simulink model "LunarMicrogridA"  (R2026b)
settings: Solver=ode23t  StopTime=simulation.timeSim  MaxStep=1/(5*solarPlant.converterSwitchingFrequency)  AbsTol=1e-3
PreLoadFcn:
  | run('LunarMicrogridA_Data');
undefined symbols (not defined in the file or in its folder): battery, bms, bmsController, boostController, connectedLoad, dcVoltage, lunarCase, maxSoC, maxVdc, minIrrad, minSoC, minVdc, olTime, sensor, solarPanel, solarPlant
libraries: fl_lib x17, nesl_utility x15, simulink x13, ee_lib x6, eePwmGenerator x3, simulink_extras x2, batteryecm_lib x1
(part 2 of 2)

== system LunarMicrogridA/PV Control/Maximum Power Point ==
  "IL " : Inport
  "Vo " : Inport  Port=2
  Vpv : Inport  Port=3
  Ipv : Inport  Port=4
  Enable : EnablePort  StatesWhenEnabling=reset
  MPPT : Subsystem
  MPPT Subsystem : Subsystem  TreatAsAtomicUnit=on
  Rate Transition : RateTransition  OutPortSampleTime=0.02
  ZOH/4 : ZeroOrderHold  SampleTime=solarPlant.timeMPPT
  Gmpp : Outport
  Vmpp : Outport  Port=2
  wires:
  ZOH/4/1 -> MPPT/2(Vpv)
  Rate Transition/1 -> MPPT/1(Ipv)
  MPPT/1(Vmpp) -> Vmpp/1, MPPT Subsystem/1(VpvRef)
  "Vo "/1 -> MPPT Subsystem/4("Vo ")
  Ipv/1 -> Rate Transition/1
  Vpv/1 -> MPPT Subsystem/2(Vpv), ZOH/4/1
  MPPT Subsystem/1(G) -> Gmpp/1
  "IL "/1 -> MPPT Subsystem/3(IL)

== system LunarMicrogridA/PV Control/PV Isolate ==
  Enable : EnablePort  StatesWhenEnabling=reset
  Constant : Constant  Value=0
  Gain : Gain
  Rate Transition : RateTransition
  Gmpp : Outport
  wires:
  Constant/1 -> Gain/1
  Gain/1 -> Rate Transition/1
  Rate Transition/1 -> Gmpp/1

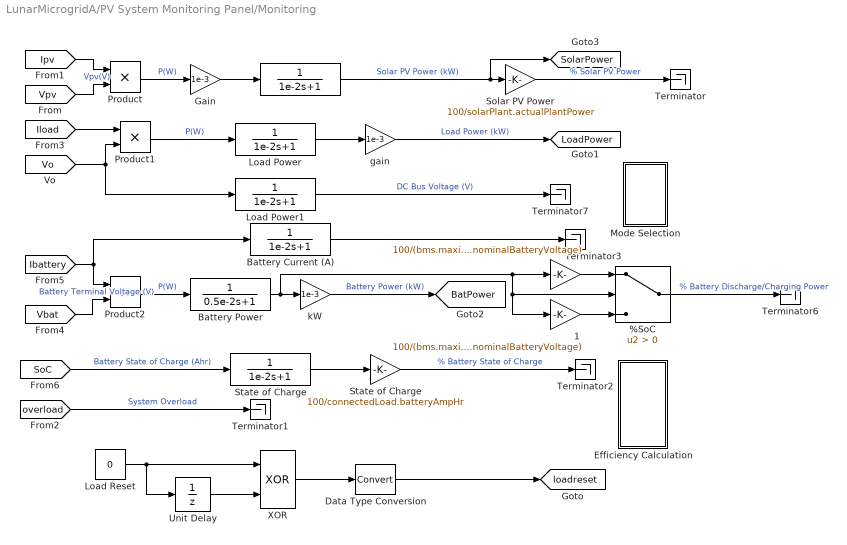
== system LunarMicrogridA/PV System Monitoring Panel/Monitoring ==
  " " : Gain  Gain=100/(bms.maximumChargingCurrentLimit*battery.nominalBatteryVoltage)
  "  " : TransferFcn  Denominator=[1e-2 1]
  " 1" : Gain  Gain=100/(bms.maximumDisChargingCurrent*battery.nominalBatteryVoltage)
  " State of Charge" : Gain  Gain=100/connectedLoad.batteryAmpHr
  %SoC : Switch  Criteria=u2 > Threshold  SaturateOnIntegerOverflow=off  InputSameDT=off
  Battery Current (A) : TransferFcn  Denominator=[1e-2 1]
  Battery Power : TransferFcn  Denominator=[0.5e-2 1]
  Data Type Conversion : DataTypeConversion  SaturateOnIntegerOverflow=off  RndMeth=Floor
  Efficiency Calculation : Subsystem
  Gain : Gain  Gain=1e-3
  Load Power : TransferFcn  Denominator=[1e-2 1]
  Load Power1 : TransferFcn  Denominator=[1e-2 1]
  Load Reset : Constant  Value=0
  Mode Selection : Subsystem
  Product : Product
  Product1 : Product
  Product2 : Product
  Solar PV Power : Gain  Gain=100/solarPlant.actualPlantPower
  State of Charge : TransferFcn  Denominator=[1e-2 1]
  Terminator{,1..3,6..7} (6 alike) : Terminator
  Unit Delay : UnitDelay  SampleTime=1e-3
  XOR : Logic  Operator=XOR  IconShape=distinctive  AllPortsSameDT=off  OutDataTypeStr=boolean
  gain : Gain  Gain=1e-3
  kW : Gain  Gain=1e-3
  tag scope: BatPower=global, LoadPower=global, SolarPower=global, loadreset=global
  wires:
  [Vpv] -> Product/2  "Vpv(V)"
  Load Power/1 -> gain/1
  Product1/1 -> Load Power/1  "P(W)"
  [Vbat] -> Product2/2  "Battery Terminal Voltage (V)"
  [Iload] -> Product1/1
  Battery Power/1 -> kW/1, " 1"/1, %SoC/2, " "/1
  "  "/1 -> [SolarPower], Solar PV Power/1  "Solar PV Power (kW)"
  [Ibattery] -> Product2/1, Battery Current (A)/1
  Product2/1 -> Battery Power/1  "P(W)"
  [Ipv] -> Product/1
  [Vo] -> Product1/2, Load Power1/1
  Product/1 -> Gain/1  "P(W)"
  [SoC] -> State of Charge/1  "Battery State of Charge (Ahr)"
  Solar PV Power/1 -> Terminator/1  "% Solar PV Power"
  gain/1 -> [LoadPower]  "Load Power (kW)"
  kW/1 -> [BatPower]  "Battery Power (kW)"
  State of Charge/1 -> " State of Charge"/1
  " State of Charge"/1 -> Terminator2/1  "% Battery State of Charge"
  " "/1 -> %SoC/1
  " 1"/1 -> %SoC/3
  %SoC/1 -> Terminator6/1  "% Battery Discharge/Charging Power"
  Battery Current (A)/1 -> Terminator3/1
  Gain/1 -> "  "/1
  Load Power1/1 -> Terminator7/1  "DC Bus Voltage (V)"
  [overload] -> Terminator1/1  "System Overload"
  XOR/1 -> Data Type Conversion/1
  Load Reset/1 -> XOR/1, Unit Delay/1
  Unit Delay/1 -> XOR/2
  Data Type Conversion/1 -> [loadreset]

== system LunarMicrogridA/Solar Plant/Solar Panel ==
  Current-Controlled Current Source : fl_lib/Electrical/Electrical Sources/Current-Controlled Current Source  K=-1*(solarPanel.numParallelCell-1)  i1_specify=off  i1_priority=None  i1=0 A  i1_nominal_specify=off  i1_nominal_value=1  i1_nominal_unit=A  i2_specify=off  i2_priority=None  i2=0 A  i2_nominal_specify=off  i2_nominal_value=1  i2_nominal_unit=A
  Solar Cell : ee_lib/Sources/Solar Cell  prm=1  Isc=solarPanel.shortCircuitCurrentPV/solarPanel.numParallelCell A  Voc=solarPanel.openCircuitVoltagePV/solarPanel.numSeriesCell V  Is=1e-6 A  Is2=0 A  Iph=7.34 A  Ir0=solarPanel.irradianceMeasurement W/m^2  ec=solarPanel.qualityFactor  N2=2  Rs=solarPanel.seriesResistance Ohm  Rp=inf Ohm  N_series=solarPanel.numSeriesCell-1  N_parallel=1  TIPH1=solarPanel.currentTemperatureCoeff 1/K  EG=1.11 eV  TXIS1=solarPanel.temperatureExponent  TXIS2=3  TRS1=0  TRP1=0  Tmeas=solarPanel.temperatureMeasurement degC  TFIXED=environment.temperature degC  thermal_mass=100 J/K  initial_temperature=25 degC
  Ir : PMIOPort  Side=Left
  + : PMIOPort  Port=2  Side=Right
  - : PMIOPort  Port=3  Side=Right
  connections:
  Current-Controlled Current Source/LConn2 -- -/RConn1 -- Solar Cell/RConn1
  Ir/RConn1 -- Solar Cell/LConn1
  Current-Controlled Current Source/LConn1 -- Solar Cell/LConn2
  Current-Controlled Current Source/RConn1 -- Current-Controlled Current Source/RConn2 -- +/RConn1

== system LunarMicrogridA/Battery Management Control/Battery Charging/Current control ==
  e : Inport
  1/T : Gain  Gain=1/bms.chargeCurrentZeroTimeConst
  Integrator : Integrator  LimitOutput=on  UpperSaturationLimit=1.3  LowerSaturationLimit=-1.3
  Kp : Gain  Gain=bms.chargeCurrentGain
  Saturation : Saturate  UpperLimit=1.5  LowerLimit=-1.5
  Sum7 : Sum  Inputs=|++
  u : Outport  VectorParamsAs1DForOutWhenUnconnected=off
  wires:
  Integrator/1 -> Sum7/2
  Saturation/1 -> u/1
  Sum7/1 -> Saturation/1
  e/1 -> Kp/1
  Kp/1 -> 1/T/1, Sum7/1
  1/T/1 -> Integrator/1

== system LunarMicrogridA/Battery Management Control/Battery Charging/Voltage control ==
  e : Inport
  1/T : Gain  Gain=1/bmsController.chosenChargeVoltageZeroTimeConst
  Integrator : Integrator  LimitOutput=on  UpperSaturationLimit=bms.maximumChargingCurrentLimit  LowerSaturationLimit=-1*bms.maximumChargingCurrentLimit
  Kp : Gain  Gain=bmsController.chosenChargeVoltageGain
  Saturation : Saturate  UpperLimit=bms.maximumChargingCurrentLimit  LowerLimit=-1*bms.maximumChargingCurrentLimit
  Sum7 : Sum  Inputs=|++
  u : Outport  VectorParamsAs1DForOutWhenUnconnected=off
  wires:
  Integrator/1 -> Sum7/2
  Saturation/1 -> u/1
  e/1 -> Kp/1
  Kp/1 -> 1/T/1, Sum7/1
  1/T/1 -> Integrator/1
  Sum7/1 -> Saturation/1

== system LunarMicrogridA/Battery Management Control/Battery Discharging/Current control ==
  e : Inport
  1/T : Gain  Gain=1/bms.dischargeCurrentZeroTimeConst
  Integrator : Integrator  InitialCondition=1  LimitOutput=on  UpperSaturationLimit=1  LowerSaturationLimit=-0.5
  Kp : Gain  Gain=bms.dischargeCurrentGain
  Saturation : Saturate  UpperLimit=1  LowerLimit=-1
  Sum7 : Sum  Inputs=|++
  u : Outport  VectorParamsAs1DForOutWhenUnconnected=off
  wires:
  Integrator/1 -> Sum7/2
  Saturation/1 -> u/1
  Sum7/1 -> Saturation/1
  e/1 -> Kp/1
  Kp/1 -> 1/T/1, Sum7/1
  1/T/1 -> Integrator/1

== system LunarMicrogridA/Battery Management Control/Battery Discharging/Voltage control ==
  e : Inport
  1/T : Gain  Gain=1/bmsController.chosenDischargeVoltageZeroTimeConst
  Integrator : Integrator  LimitOutput=on  UpperSaturationLimit=bms.maximumDisChargingCurrent  LowerSaturationLimit=-1*bms.maximumDisChargingCurrent
  Kp : Gain  Gain=bmsController.chosenDischargeVoltageGain
  Saturation : Saturate  UpperLimit=bms.maximumDisChargingCurrent  LowerLimit=-1*bms.maximumDisChargingCurrent
  Sum7 : Sum  Inputs=|++
  u : Outport  VectorParamsAs1DForOutWhenUnconnected=off
  wires:
  Integrator/1 -> Sum7/2
  Saturation/1 -> u/1
  e/1 -> Kp/1
  Kp/1 -> 1/T/1, Sum7/1
  1/T/1 -> Integrator/1
  Sum7/1 -> Saturation/1

== system LunarMicrogridA/PV Control/Constant Voltage/Current control ==
  e : Inport
  Integrator : Integrator  LimitOutput=on  UpperSaturationLimit=1.5  LowerSaturationLimit=-1.5
  Ki : Gain  Gain=1/boostController.mppCurrentZeroTimeConst
  Kp : Gain  Gain=boostController.mppCurrentGain
  Saturation : Saturate  UpperLimit=1.5  LowerLimit=-1.5
  Sum7 : Sum  Inputs=|++
  u : Outport  VectorParamsAs1DForOutWhenUnconnected=off
  wires:
  Integrator/1 -> Sum7/2
  Saturation/1 -> u/1
  Sum7/1 -> Saturation/1
  e/1 -> Kp/1
  Kp/1 -> Ki/1, Sum7/1
  Ki/1 -> Integrator/1

== system LunarMicrogridA/PV Control/Constant Voltage/Voltage control ==
  e : Inport
  1/T : Gain  Gain=1/boostController.mppVoltageZeroTimeConst
  Integrator : Integrator  LimitOutput=on  UpperSaturationLimit=boostController.mppVoltageLoopMax  LowerSaturationLimit=boostController.mppVoltageLoopMin
  Kp : Gain  Gain=boostController.mppVoltageGain
  Saturation : Saturate  UpperLimit=boostController.mppVoltageLoopMax  LowerLimit=boostController.mppVoltageLoopMin
  Sum7 : Sum  Inputs=|++
  u : Outport  VectorParamsAs1DForOutWhenUnconnected=off
  wires:
  Integrator/1 -> Sum7/2
  Saturation/1 -> u/1
  Sum7/1 -> Saturation/1
  e/1 -> Kp/1
  Kp/1 -> 1/T/1, Sum7/1
  1/T/1 -> Integrator/1

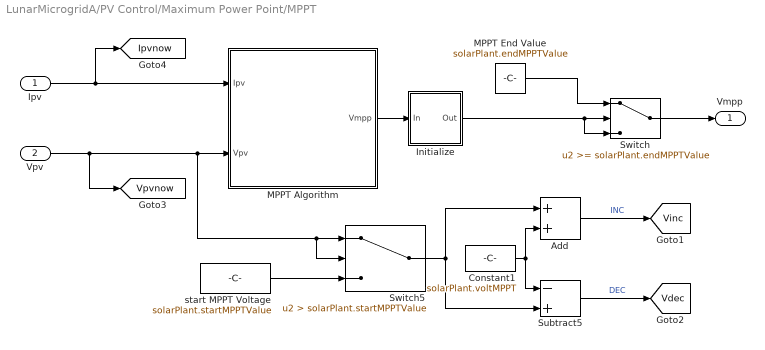
== system LunarMicrogridA/PV Control/Maximum Power Point/MPPT ==
  Ipv : Inport
  Vpv : Inport  Port=2
  Add : Sum
  Constant1 : Constant  Value=solarPlant.voltMPPT
  Initialize : Subsystem
  MPPT Algorithm : Subsystem  Variant=on
  MPPT End Value : Constant  Value=solarPlant.endMPPTValue
  Subtract5 : Sum  Inputs=-+
  Switch : Switch  Threshold=solarPlant.endMPPTValue  SaturateOnIntegerOverflow=off  InputSameDT=off
  Switch5 : Switch  Criteria=u2 > Threshold  Threshold=solarPlant.startMPPTValue  SaturateOnIntegerOverflow=off  InputSameDT=off
  start MPPT Voltage : Constant  Value=solarPlant.startMPPTValue
  Vmpp : Outport  VectorParamsAs1DForOutWhenUnconnected=off
  tag scope: Ipvnow=global, Vdec=global, Vinc=global, Vpvnow=global
  wires:
  Switch5/1 -> Add/1, Subtract5/2
  Add/1 -> [Vinc]  "INC"
  start MPPT Voltage/1 -> Switch5/3
  Vpv/1 -> [Vpvnow], Switch5/2, Switch5/1, MPPT Algorithm/2(Vpv)
  Constant1/1 -> Add/2, Subtract5/1
  Subtract5/1 -> [Vdec]  "DEC"
  Ipv/1 -> [Ipvnow], MPPT Algorithm/1(Ipv)
  MPPT Algorithm/1(Vmpp) -> Initialize/1(In)
  Initialize/1(Out) -> Switch/3, Switch/2
  Switch/1 -> Vmpp/1
  MPPT End Value/1 -> Switch/1

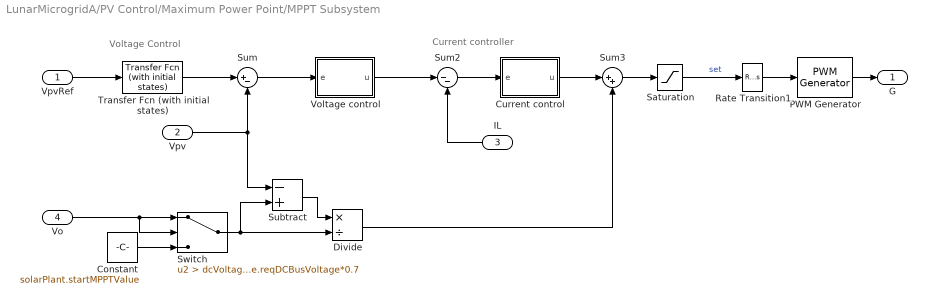
== system LunarMicrogridA/PV Control/Maximum Power Point/MPPT Subsystem ==
  note: Current controller
  note: Voltage Control
  VpvRef : Inport
  Vpv : Inport  Port=2
  IL : Inport  Port=3
  "Vo " : Inport  Port=4
  Constant : Constant  Value=solarPlant.startMPPTValue
  Current control : Subsystem
  Divide : Product  Inputs=*/
  PWM Generator : eePwmGenerator/PWM Generator  CarrCount=Up  Tper=1/solarPlant.converterSwitchingFrequency  Tdelay=0  Ts=1/(10*solarPlant.converterSwitchingFrequency)
  Rate Transition1 : RateTransition  OutPortSampleTime=1/(10*solarPlant.converterSwitchingFrequency)
  Saturation : Saturate  UpperLimit=1  LowerLimit=0
  Subtract : Sum  Inputs=-+
  Sum : Sum  Inputs=|+-
  Sum2 : Sum  Inputs=|--
  Sum3 : Sum  Inputs=|++
  Switch : Switch  Criteria=u2 > Threshold  Threshold=dcVoltage.reqDCBusVoltage*0.7  SaturateOnIntegerOverflow=off  InputSameDT=off
  Transfer Fcn (with initial states) : simulink_extras/Additional Linear/Transfer Fcn (with initial states)  N=[1]  D=[0.00001 1]  X0=solarPlant.startMPPTValue
  Voltage control : Subsystem
  G : Outport
  wires:
  Subtract/1 -> Divide/1
  Voltage control/1(u) -> Sum2/1
  Current control/1(u) -> Sum3/1
  Sum2/1 -> Current control/1(e)
  "Vo "/1 -> Switch/2, Switch/1
  VpvRef/1 -> Transfer Fcn (with initial states)/1
  Constant/1 -> Switch/3
  Switch/1 -> Divide/2, Subtract/2
  Vpv/1 -> Subtract/1, Sum/2
  Saturation/1 -> Rate Transition1/1  "set"
  Rate Transition1/1 -> PWM Generator/1
  PWM Generator/1 -> G/1
  Divide/1 -> Sum3/2
  Sum/1 -> Voltage control/1(e)
  IL/1 -> Sum2/2
  Transfer Fcn (with initial states)/1 -> Sum/1
  Sum3/1 -> Saturation/1

== system LunarMicrogridA/PV System Monitoring Panel/Monitoring/Efficiency Calculation ==
  Abs : Abs  SaturateOnIntegerOverflow=off
  Add : Sum
  Add1 : Sum
  Constant : Constant  Value=100e3
  Constant1 : Constant  Value=100e3
  Divide : Product  Inputs=/*
  Divide1 : Product  Inputs=/*
  Gain : Gain  Gain=100
  Switch : Switch  Criteria=u2 > Threshold  SaturateOnIntegerOverflow=off  InputSameDT=off
  Switch1 : Switch  Criteria=u2 > Threshold  SaturateOnIntegerOverflow=off  InputSameDT=off
  Switch2 : Switch  Criteria=u2 > Threshold  SaturateOnIntegerOverflow=off  InputSameDT=off
  Terminator : Terminator
  wires:
  [BatPower] -> Abs/1, Add/2, Switch/2
  [LoadPower] -> Add/1
  [SolarPower] -> Switch1/1, Switch1/2, Add1/2
  Constant/1 -> Switch1/3
  Switch1/1 -> Divide/1
  Add/1 -> Divide/2
  Abs/1 -> Add1/1
  [LoadPower] -> Divide1/2
  Add1/1 -> Switch2/2, Switch2/1
  Constant1/1 -> Switch2/3
  Switch2/1 -> Divide1/1
  Divide/1 -> Switch/1
  Divide1/1 -> Switch/3
  Switch/1 -> Gain/1
  Gain/1 -> Terminator/1  "% Efficiency"

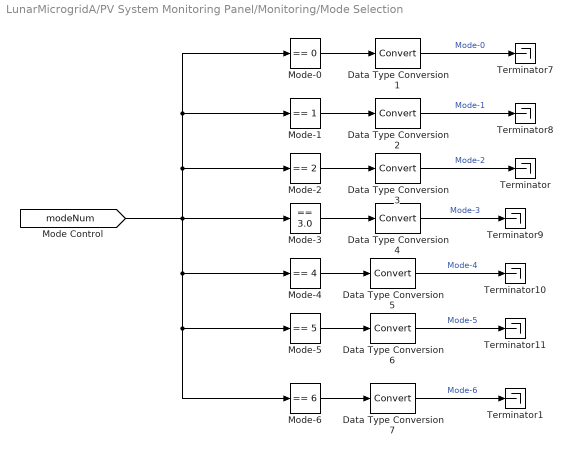
== system LunarMicrogridA/PV System Monitoring Panel/Monitoring/Mode Selection ==
  Data Type Conversion{1..7} (7 alike) : DataTypeConversion  SaturateOnIntegerOverflow=off  RndMeth=Floor
  Mode-0 : simulink/Logic and Bit Operations/Compare To Constant  relop===  const=0  OutDataTypeStr=boolean
  Mode-1 : simulink/Logic and Bit Operations/Compare To Constant  relop===  const=1  OutDataTypeStr=boolean
  Mode-2 : simulink/Logic and Bit Operations/Compare To Constant  relop===  const=2  OutDataTypeStr=boolean
  Mode-3 : simulink/Logic and Bit Operations/Compare To Constant  relop===  const=3.0  OutDataTypeStr=boolean
  Mode-4 : simulink/Logic and Bit Operations/Compare To Constant  relop===  const=4  OutDataTypeStr=boolean
  Mode-5 : simulink/Logic and Bit Operations/Compare To Constant  relop===  const=5  OutDataTypeStr=boolean
  Mode-6 : simulink/Logic and Bit Operations/Compare To Constant  relop===  const=6  OutDataTypeStr=boolean
  Terminator{,1,7..11} (7 alike) : Terminator
  wires:
  Mode-0/1 -> Data Type Conversion1/1
  Mode-3/1 -> Data Type Conversion4/1
  [modeNum] -> Mode-3/1, Mode-4/1, Mode-5/1, Mode-6/1, Mode-2/1, Mode-1/1, Mode-0/1
  Mode-4/1 -> Data Type Conversion5/1
  Mode-1/1 -> Data Type Conversion2/1
  Mode-2/1 -> Data Type Conversion3/1
  Mode-5/1 -> Data Type Conversion6/1
  Mode-6/1 -> Data Type Conversion7/1
  Data Type Conversion1/1 -> Terminator7/1  "Mode-0"
  Data Type Conversion2/1 -> Terminator8/1  "Mode-1"
  Data Type Conversion3/1 -> Terminator/1  "Mode-2"
  Data Type Conversion4/1 -> Terminator9/1  "Mode-3"
  Data Type Conversion5/1 -> Terminator10/1  "Mode-4"
  Data Type Conversion6/1 -> Terminator11/1  "Mode-5"
  Data Type Conversion7/1 -> Terminator1/1  "Mode-6"

== system LunarMicrogridA/PV Control/Maximum Power Point/MPPT/Initialize ==
  In : Inport
  Constant : Constant  Value=solarPlant.startMPPTValue
  Constant2 : Constant
  Integrator : Integrator
  Switch1 : Switch  Criteria=u2 > Threshold  Threshold=solarPlant.startMPPTValue  SaturateOnIntegerOverflow=off  InputSameDT=off
  Switch2 : Switch  Criteria=u2 > Threshold  Threshold=solarPlant.timeMPPT  SaturateOnIntegerOverflow=off  InputSameDT=off
  Out : Outport
  wires:
  Constant/1 -> Switch1/3
  Switch1/1 -> Switch2/1
  In/1 -> Switch1/2, Switch1/1
  Switch2/1 -> Out/1
  Constant2/1 -> Integrator/1
  [Vpvnow] -> Switch2/3
  Integrator/1 -> Switch2/2

== system LunarMicrogridA/PV Control/Maximum Power Point/MPPT/MPPT Algorithm ==
  Ipv : Inport
  Vpv : Inport  Port=2
  IncrementalConductance : Subsystem  VariantControl=incrementalConductance
  PerturbationAndObsrvation : Subsystem  VariantControl=perturbationAndObservation
  Vmpp : Outport  VectorParamsAs1DForOutWhenUnconnected=off

== system LunarMicrogridA/PV Control/Maximum Power Point/MPPT Subsystem/Current control ==
  e : Inport
  Integrator : Integrator  InitialCondition=1  LimitOutput=on  UpperSaturationLimit=1  LowerSaturationLimit=-0.5
  Ki : Gain  Gain=1/boostController.mppCurrentZeroTimeConst
  Kp : Gain  Gain=boostController.mppCurrentGain
  Saturation : Saturate  UpperLimit=1  LowerLimit=-0.3
  Sum7 : Sum  Inputs=|++
  u : Outport  VectorParamsAs1DForOutWhenUnconnected=off
  wires:
  Integrator/1 -> Sum7/2
  Saturation/1 -> u/1
  Sum7/1 -> Saturation/1
  e/1 -> Kp/1
  Kp/1 -> Ki/1, Sum7/1
  Ki/1 -> Integrator/1

== system LunarMicrogridA/PV Control/Maximum Power Point/MPPT Subsystem/Voltage control ==
  e : Inport
  1/T : Gain  Gain=1/boostController.mppVoltageZeroTimeConst
  Integrator : Integrator  LimitOutput=on  UpperSaturationLimit=boostController.mppVoltageLoopMax  LowerSaturationLimit=boostController.mppVoltageLoopMin
  Kp : Gain  Gain=boostController.mppVoltageGain
  Saturation : Saturate  UpperLimit=boostController.mppVoltageLoopMax  LowerLimit=boostController.mppVoltageLoopMin
  Sum7 : Sum  Inputs=|++
  u : Outport  VectorParamsAs1DForOutWhenUnconnected=off
  wires:
  Integrator/1 -> Sum7/2
  Saturation/1 -> u/1
  Sum7/1 -> Saturation/1
  e/1 -> Kp/1
  Kp/1 -> 1/T/1, Sum7/1
  1/T/1 -> Integrator/1

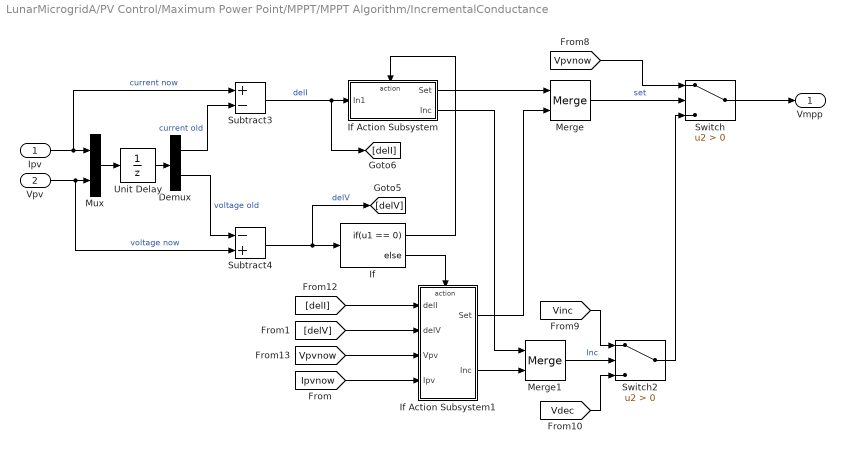
== system LunarMicrogridA/PV Control/Maximum Power Point/MPPT/MPPT Algorithm/IncrementalConductance ==
  Ipv : Inport
  Vpv : Inport  Port=2
  Demux : Demux  Outputs=2
  If : If  IfExpression=u1 == 0
  If Action Subsystem : Subsystem  TreatAsAtomicUnit=on
  If Action Subsystem1 : Subsystem  TreatAsAtomicUnit=on
  Merge : Merge
  Merge1 : Merge
  Mux : Mux  Inputs=2
  Subtract3 : Sum  Inputs=+-
  Subtract4 : Sum  Inputs=-+
  Switch : Switch  Criteria=u2 > Threshold  SaturateOnIntegerOverflow=off  InputSameDT=off
  Switch2 : Switch  Criteria=u2 > Threshold  SaturateOnIntegerOverflow=off  InputSameDT=off
  Unit Delay : UnitDelay  InitialCondition=solarPlant.startMPPTValue  SampleTime=solarPlant.timeMPPT
  Vmpp : Outport  VectorParamsAs1DForOutWhenUnconnected=off
  wires:
  Merge1/1 -> Switch2/2  "Inc"
  [Vpvnow] -> Switch/1
  If Action Subsystem1/2(Inc) -> Merge1/2
  If Action Subsystem/2(Inc) -> Merge1/1
  If/2 -> If Action Subsystem1/Action
  If Action Subsystem/1(Set) -> Merge/1
  [delV] -> If Action Subsystem1/2(delV)
  [delI] -> If Action Subsystem1/1(delI)
  Merge/1 -> Switch/2  "set"
  If Action Subsystem1/1(Set) -> Merge/2
  If/1 -> If Action Subsystem/Action
  [Vpvnow] -> If Action Subsystem1/3(Vpv)
  Switch2/1 -> Switch/3
  [Ipvnow] -> If Action Subsystem1/4(Ipv)
  Ipv/1 -> Mux/1, Subtract3/1  "current now"
  Unit Delay/1 -> Demux/1
  Mux/1 -> Unit Delay/1
  Vpv/1 -> Subtract4/2, Mux/2  "voltage now"
  Demux/2 -> Subtract4/1  "voltage old"
  Demux/1 -> Subtract3/2  "current old"
  Subtract3/1 -> [delI], If Action Subsystem/1(In1)  "delI"
  Subtract4/1 -> [delV], If/1  "delV"
  Switch/1 -> Vmpp/1
  [Vdec] -> Switch2/3
  [Vinc] -> Switch2/1

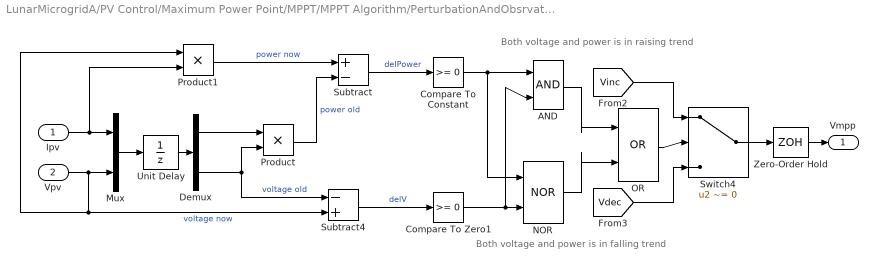
== system LunarMicrogridA/PV Control/Maximum Power Point/MPPT/MPPT Algorithm/PerturbationAndObsrvation ==
  note: Both voltage and power is in falling trend
  note: Both voltage and power is in raising trend
  Ipv : Inport
  Vpv : Inport  Port=2
  AND : Logic  IconShape=distinctive  AllPortsSameDT=off  OutDataTypeStr=boolean
  Compare To Constant : simulink/Logic and Bit Operations/Compare To Constant  relop=>=  const=0  OutDataTypeStr=boolean
  Compare To Zero1 : simulink/Logic and Bit Operations/Compare To Zero  relop=>=  OutDataTypeStr=boolean
  Demux : Demux  Outputs=2
  Mux : Mux  Inputs=2
  NOR : Logic  Operator=NOR  IconShape=distinctive  AllPortsSameDT=off  OutDataTypeStr=boolean
  OR : Logic  Operator=OR  IconShape=distinctive  AllPortsSameDT=off  OutDataTypeStr=boolean
  Product : Product
  Product1 : Product
  Subtract : Sum  Inputs=+-
  Subtract4 : Sum  Inputs=-+
  Switch4 : Switch  Criteria=u2 ~= 0  SaturateOnIntegerOverflow=off  InputSameDT=off
  Unit Delay : UnitDelay  InitialCondition=solarPlant.startMPPTValue  SampleTime=solarPlant.timeMPPT
  Zero-Order Hold : ZeroOrderHold  SampleTime=solarPlant.timeMPPT
  Vmpp : Outport  VectorParamsAs1DForOutWhenUnconnected=off
  wires:
  NOR/1 -> OR/2
  OR/1 -> Switch4/2
  Compare To Zero1/1 -> AND/2, NOR/2
  AND/1 -> OR/1
  Compare To Constant/1 -> AND/1, NOR/1
  Mux/1 -> Unit Delay/1
  Ipv/1 -> Product1/2, Mux/1
  Demux/1 -> Product/1
  Unit Delay/1 -> Demux/1
  Demux/2 -> Product/2, Subtract4/1  "voltage old"
  Vpv/1 -> Subtract4/2, Product1/1, Mux/2  "voltage now"
  Product1/1 -> Subtract/1  "power now"
  Product/1 -> Subtract/2  "power old"
  Subtract4/1 -> Compare To Zero1/1  "delV"
  Subtract/1 -> Compare To Constant/1  "delPower"
  Switch4/1 -> Zero-Order Hold/1
  [Vdec] -> Switch4/3
  [Vinc] -> Switch4/1
  Zero-Order Hold/1 -> Vmpp/1

== system LunarMicrogridA/PV Control/Maximum Power Point/MPPT/MPPT Algorithm/IncrementalConductance/If Action Subsystem ==
  In1 : Inport
  Action Port : ActionPort  ActionPortLabel=if(u1 == 0)
  Compare To Constant : simulink/Logic and Bit Operations/Compare To Constant  relop===  const=0  OutDataTypeStr=boolean
  Compare To Zero2 : simulink/Logic and Bit Operations/Compare To Zero  relop=>  OutDataTypeStr=boolean
  Set : Outport  VectorParamsAs1DForOutWhenUnconnected=off
  Inc : Outport  Port=2  VectorParamsAs1DForOutWhenUnconnected=off
  wires:
  Compare To Constant/1 -> Set/1  "Yes"
  Compare To Zero2/1 -> Inc/1  "Yes"
  In1/1 -> Compare To Zero2/1, Compare To Constant/1  "delI"

== system LunarMicrogridA/PV Control/Maximum Power Point/MPPT/MPPT Algorithm/IncrementalConductance/If Action Subsystem1 ==
  delI : Inport
  delV : Inport  Port=2
  Vpv : Inport  Port=3
  Ipv : Inport  Port=4
  Action Port : ActionPort  ActionPortLabel=else
  Add : Sum
  Compare To Zero : simulink/Logic and Bit Operations/Compare To Zero  relop===  OutDataTypeStr=boolean
  Compare To Zero1 : simulink/Logic and Bit Operations/Compare To Zero  relop=>  OutDataTypeStr=boolean
  Divide : Product  Inputs=*/
  Product : Product
  Set : Outport  VectorParamsAs1DForOutWhenUnconnected=off
  Inc : Outport  Port=2  VectorParamsAs1DForOutWhenUnconnected=off
  wires:
  delI/1 -> Divide/1
  delV/1 -> Divide/2
  Divide/1 -> Product/1
  Add/1 -> Compare To Zero1/1, Compare To Zero/1
  Compare To Zero/1 -> Set/1  "set"
  Vpv/1 -> Product/2
  Product/1 -> Add/1
  Ipv/1 -> Add/2
  Compare To Zero1/1 -> Inc/1  "Increase"

== stateflow chart LunarMicrogridA/Mode Control ==
  state Mode2_BatCharge_pvMPPT
    entry:
    pvMPPT=1;
    BatCharge=1;
    modeNum=2;
    overload=0;
    exit:
    pvMPPT=0; BatCharge=0;
  state Start_Mode
    entry:
    ShutDown = 0;
    loadShutDown = 1;
    pvMPPT=0;
    VoltageControl=1;
    BatIsolate=1;
    modeNum=0;
    overload=0;
    exit:
    pvMPPT=0;
    BatIsolate=0;
    VoltageControl=0;
    loadShutDown = 0;
  state Mode5_System_ShutDown
    entry:
    PVoff=1; BatIsolate=1;
    ShutDown =1; modeNum=5;
    exit:
    ShutDown =0; PVoff=0;
    BatIsolate=0;
  state Mode1_batIsolated_pvVoltControl
    entry:
    VoltageControl=1; BatIsolate=1;
    modeNum=1;
    exit:
    VoltageControl=0; BatIsolate=0;
  state Mode6_pvMPPT_BatCharge_noload
    entry:
    pvMPPT=1; BatCharge=1;
    loadShutDown=1; modeNum=6;
    overload=1;
    exit:
    loadShutDown=0; pvMPPT=0;
    BatCharge=0;
  state Mode3_BatDischarge_pvMPPT
    entry:
    pvMPPT=1; BatDischarge=1;
    modeNum=3; overload=0;
    exit:
    pvMPPT=0;  BatDischarge=0;
  state Mode4_night_mode
    entry:
    PVoff=1; BatDischarge=1;
    modeNum=4;
    exit:
    PVoff=0; BatDischarge=0;
  Mode2_BatCharge_pvMPPT -> (junction 121) [order 3] : [Irrad<minIrrad && SoC>minSoC]
  Mode2_BatCharge_pvMPPT -> (junction 131) [order 2] : [Vdc < minVdc && SoC>minSoC]
  (junction 121) -> Mode4_night_mode
  (junction 131) -> (junction 154)
  Mode2_BatCharge_pvMPPT -> (junction 117) [order 5] : [Irrad<minIrrad && SoC<minSoC]
  (junction 132) -> Mode2_BatCharge_pvMPPT : [Vdc > maxVdc && Irrad>minIrrad]
  (junction 117) -> Mode5_System_ShutDown
  (junction 155) -> (junction 132)
  (junction 130) -> Mode2_BatCharge_pvMPPT : [(Irrad >minIrrad && overload==0) || ...
      | (overload==1 && rsflag==1)]
  Mode5_System_ShutDown -> (junction 130)
  Start_Mode -> Mode2_BatCharge_pvMPPT [order 1] : [SoC<minSoC]
  (junction 123) -> Mode2_BatCharge_pvMPPT
  Mode6_pvMPPT_BatCharge_noload -> (junction 123) [order 3] : [rsflag ==1 && Irrad > minIrrad  ...
      | && SoC <= minSoC]
  Mode2_BatCharge_pvMPPT -> (junction 125) [order 4]
  (default) -> Start_Mode
  (junction 125) -> Mode6_pvMPPT_BatCharge_noload : [duration(Vdc<minVdc)>olTime ...
      |  && SoC<minSoC]
  Mode2_BatCharge_pvMPPT -> Mode1_batIsolated_pvVoltControl [order 1] : [(SoC>maxSoC) || ...
      | (duration(Vdc>maxVdc)>olTime)]
  Start_Mode -> Mode3_BatDischarge_pvMPPT [order 2] : [SoC>minSoC]
  Mode1_batIsolated_pvVoltControl -> (junction 126)
  Mode6_pvMPPT_BatCharge_noload -> Mode5_System_ShutDown [order 2] : [(SoC<minSoC && ...
      | Irrad<minIrrad)|| ...
      | SoC>maxSoC]
  (junction 126) -> Mode3_BatDischarge_pvMPPT : [Vdc<minVdc]
  (junction 161) -> Mode5_System_ShutDown
  Mode4_night_mode -> Mode5_System_ShutDown [order 2] : [SoC<minSoC]
  Mode6_pvMPPT_BatCharge_noload -> (junction 127) [order 1] : [SoC>minSoC && rsflag==1]
  (junction 127) -> Mode3_BatDischarge_pvMPPT
  (junction 133) -> Mode6_pvMPPT_BatCharge_noload
  Mode3_BatDischarge_pvMPPT -> (junction 133) [order 2] : [(duration(Vdc<minVdc)>olTime || ...
      |  (SoC<minSoC && Vdc<minVdc)) && Irrad>minIrrad]
  Mode3_BatDischarge_pvMPPT -> (junction 161) [order 3] : [(SoC<minSoC && Irrad<minIrrad) || ( Irrad<minIrrad && duration(Vdc<minVdc)>olTime) ]
  Mode3_BatDischarge_pvMPPT -> (junction 155) [order 1]
  Mode4_night_mode -> Mode3_BatDischarge_pvMPPT [order 1] : [Irrad>minIrrad]
  Mode3_BatDischarge_pvMPPT -> Mode4_night_mode [order 4] : [Irrad<minIrrad && SoC>minSoC]
  (junction 154) -> Mode3_BatDischarge_pvMPPT
  data: Irrad input; Vdc input; SoC input; ShutDown output; maxSoC parameter; maxVdc parameter; minIrrad parameter; minSoC parameter; minVdc parameter; loadShutDown output; VoltageControl output; data output; BatCharge output; BatDischarge output; BatIsolate output; PVoff output; pvMPPT output; modeNum output; rsflag input; overload output; olTime parameter
